simulink subsystem "BEVController_Basic_refsub"  (R2026a)
settings: Solver=VariableStepAuto
undefined symbols (not defined in the file or in its folder): bevControl
settings Model: Creator=isaacito  LastModifiedBy=isaacito

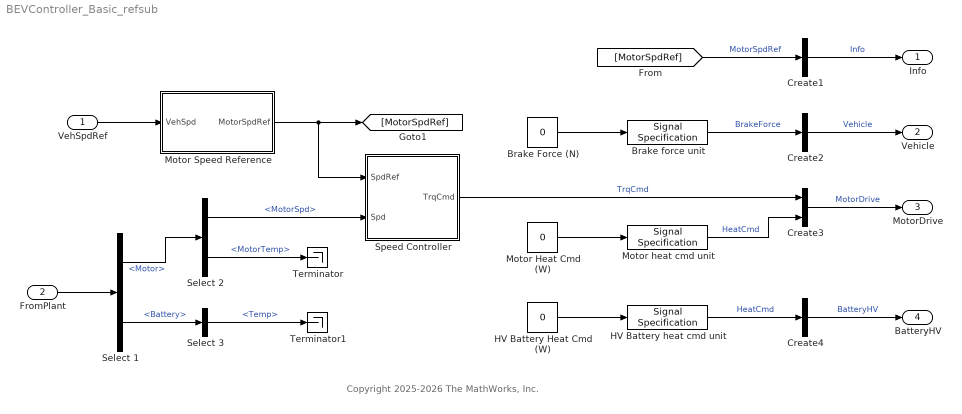
== system BEVController_Basic_refsub ==
  note: Copyright 2025-2026 The MathWorks, Inc.
  VehSpdRef : Inport
  FromPlant : Inport  Port=2
  Brake Force (N) : Constant  Value=0
  Brake force unit : SignalSpecification  Unit=N
  Create1 : BusCreator  Inputs=1
  Create2 : BusCreator  Inputs=1
  Create3 : BusCreator  Inputs=2
  Create4 : BusCreator  Inputs=1
  HV Battery Heat Cmd (W) : Constant  Value=0
  HV Battery heat cmd unit : SignalSpecification  Unit=W
  Motor Heat Cmd (W) : Constant  Value=0
  Motor Speed Reference : Subsystem
  Motor heat cmd unit : SignalSpecification  Unit=W
  Select 1 : BusSelector  OutputSignals=Motor,Battery
  Select 2 : BusSelector  OutputSignals=MotorSpd,MotorTemp
  Select 3 : BusSelector  OutputSignals=Temp
  Speed Controller : Subsystem
      settings: PortSchema="{\"entries\":[{\"content\":{\"sides\":[{\"content\":{\"connectorIds\":[\"Out1\"]},\"type\":\"ConnectorPlacement.EquallySpacedRectSide\",\"uuid\":\"12b9f2c9-2b28-451b-ad36-7fe4150db485\"},{\"content\":{\"connectorIds\":[\"In1\",\"In2\"],\"side\":\"RIGHT\"},\"type\":\"ConnectorPlacement.EquallySpacedRectSide\",\"uuid\":\"c0fdf9a4-483a-4ddc-b663-6299fcc79327\"},{\"content\":{\"connectorIds\":[],\"side\":\"TOP\"},\"type\":\"ConnectorPlacement.EquallySpacedRectSide\",\"uuid\":\"3f20082e-8487-45e3-9fd7-d6d75741df4d\"}]},\"type\":\"ConnectorPlacement.EquallySpacedConnector\",\"uuid\":\"9361cdd3-74d8-46ee-ae7f-e2dde5d31ed1\"}],\"packageUris\":[\"http://schema.mathworks.com/mf0/Connector/R2020b\"],\"version\":\"1.0\"}"
  Terminator : Terminator
  Terminator1 : Terminator
  Info : Outport
  Vehicle : Outport  Port=2
  MotorDrive : Outport  Port=3
  BatteryHV : Outport  Port=4
  wires:
  Motor Speed Reference/1(MotorSpdRef) -> [MotorSpdRef], Speed Controller/1(SpdRef)
  Select 2/1 -> Speed Controller/2(Spd)  "<MotorSpd>"
  Speed Controller/1(TrqCmd) -> Create3/1  "TrqCmd"
  VehSpdRef/1 -> Motor Speed Reference/1(VehSpd)
  Brake Force (N)/1 -> Brake force unit/1
  FromPlant/1 -> Select 1/1
  Select 1/1 -> Select 2/1  "<Motor>"
  Create1/1 -> Info/1  "Info"
  Create2/1 -> Vehicle/1  "Vehicle"
  Create3/1 -> MotorDrive/1  "MotorDrive"
  Create4/1 -> BatteryHV/1  "BatteryHV"
  Select 1/2 -> Select 3/1  "<Battery>"
  Motor Heat Cmd (W)/1 -> Motor heat cmd unit/1
  HV Battery Heat Cmd (W)/1 -> HV Battery heat cmd unit/1
  Select 2/2 -> Terminator/1  "<MotorTemp>"
  Select 3/1 -> Terminator1/1  "<Temp>"
  Motor heat cmd unit/1 -> Create3/2  "HeatCmd"
  HV Battery heat cmd unit/1 -> Create4/1  "HeatCmd"
  Brake force unit/1 -> Create2/1  "BrakeForce"
  [MotorSpdRef] -> Create1/1  "MotorSpdRef"

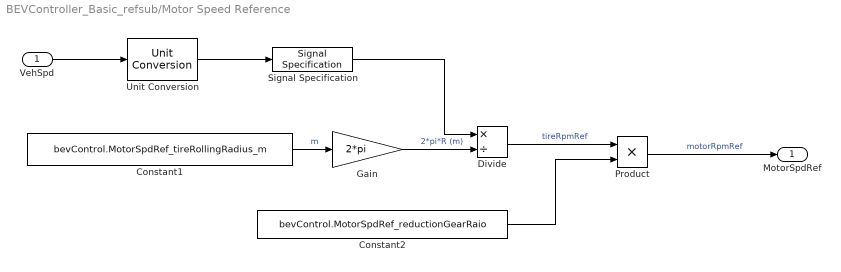
== system BEVController_Basic_refsub/Motor Speed Reference ==
  VehSpd : Inport  Unit=km/hr
  Constant1 : Constant  Value=bevControl.MotorSpdRef_tireRollingRadius_m
  Constant2 : Constant  Value=bevControl.MotorSpdRef_reductionGearRaio
  Divide : Product  Inputs=*/
  Gain : Gain  Gain=2*pi
  Product : Product
  Signal Specification : SignalSpecification  Unit=m/min
  Unit Conversion : UnitConversion
  MotorSpdRef : Outport  Unit=rpm  VectorParamsAs1DForOutWhenUnconnected=off
  wires:
  Constant1/1 -> Gain/1  "m"
  Product/1 -> MotorSpdRef/1  "motorRpmRef"
  Constant2/1 -> Product/2
  Divide/1 -> Product/1  "tireRpmRef"
  Gain/1 -> Divide/2  "2*pi*R (m)"
  Signal Specification/1 -> Divide/1
  Unit Conversion/1 -> Signal Specification/1
  VehSpd/1 -> Unit Conversion/1

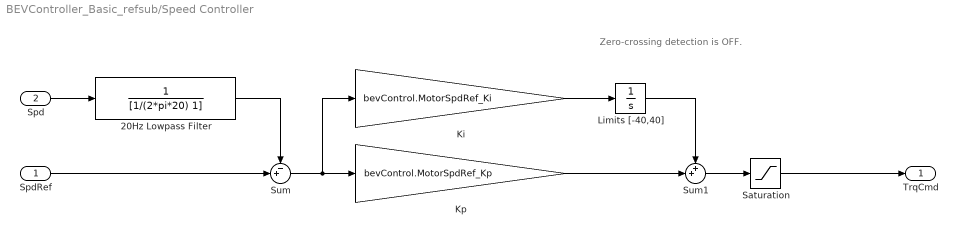
== system BEVController_Basic_refsub/Speed Controller ==
  note: Zero-crossing detection is OFF.
  SpdRef : Inport  Unit=rpm
      settings: AttributesFormatString=%<Unit>
  Spd : Inport  Port=2  Unit=rpm
      settings: AttributesFormatString=%<Unit>
  20Hz Lowpass Filter : TransferFcn  Denominator=[1/(2*pi*20) 1]
  Ki : Gain  Gain=bevControl.MotorSpdRef_Ki
  Kp : Gain  Gain=bevControl.MotorSpdRef_Kp
  Limits [-40,40] : Integrator  LimitOutput=on  UpperSaturationLimit=40  LowerSaturationLimit=-40  ZeroCross=off
  Saturation : Saturate  UpperLimit=bevControl.MotorDriveUnit_trqMax_Nm  LowerLimit=-bevControl.MotorDriveUnit_trqMax_Nm
      settings: AttributesFormatString=|
      | %<UpperLimit>
      | %<LowerLimit>
  Sum : Sum  Inputs=-+|
  Sum1 : Sum  Inputs=++|
  TrqCmd : Outport  Unit=N*m  VectorParamsAs1DForOutWhenUnconnected=off
      settings: AttributesFormatString=%<Unit>
  wires:
  SpdRef/1 -> Sum/2
  Spd/1 -> 20Hz Lowpass Filter/1
  Sum1/1 -> Saturation/1
  Sum/1 -> Ki/1, Kp/1
  Ki/1 -> Limits [-40,40]/1
  Kp/1 -> Sum1/2
  Limits [-40,40]/1 -> Sum1/1
  20Hz Lowpass Filter/1 -> Sum/1
  Saturation/1 -> TrqCmd/1
